simulink library "sf_pole_vault_lib"  (R2025b)
settings: Solver=VariableStepAuto  StartTime=0.0  StopTime=10.0  RelTol=1e-3
undefined symbols (not defined in the file or in its folder): theta0
libraries: simulink_extras x3
settings Model: Creator=The MathWorks, Inc.  LastModifiedBy=The MathWorks, Inc.
settings SolverCC: AlgebraicLoopSolver=TrustRegion
settings DataIOCC: ReturnWorkspaceOutputs=off
settings OptimizationCC: ReuseModelBlockBuffer=off
settings DebuggingCC: UnconnectedInputMsg=warning  UnconnectedOutputMsg=warning  UnconnectedLineMsg=warning  ArithmeticOperatorsInVariantConditions=warning
settings ModelReferenceCC: EnableRefExpFcnMdlSchedulingChecks=on
settings SFSimCC: SimUseLocalCustomCode=off  CustomCodeUndefinedFunction=UseInterfaceOnly
settings RTWCC: RTWUseLocalCustomCode=off  GPUComputeCapability=3.5

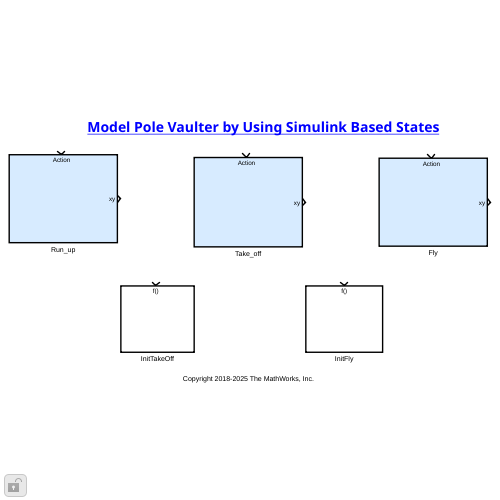
[thumbnail: Simulink's stored preview of the top-level diagram]
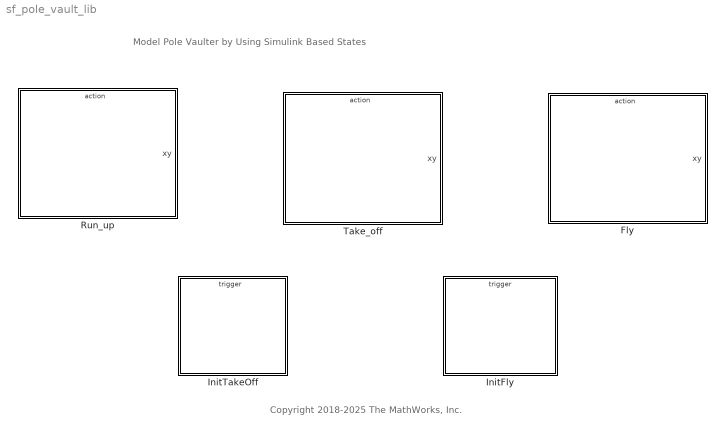
== system sf_pole_vault_lib ==
  note: Copyright 2018-2025 The MathWorks, Inc.
  note: Model Pole Vaulter by Using Simulink Based States
  Fly : Subsystem
      settings: UndoDeleteFcn=Stateflow.SLINSF.SimulinkMan.restorePreDeleteFcn  PreDeleteFcn=Stateflow.SLINSF.SimulinkMan.removePreDeleteFcn
  InitFly : Subsystem
      settings: UndoDeleteFcn=Stateflow.SLINSF.SimulinkMan.restorePreDeleteFcn  PreDeleteFcn=Stateflow.SLINSF.SimulinkMan.removePreDeleteFcn
  InitTakeOff : Subsystem
      settings: UndoDeleteFcn=Stateflow.SLINSF.SimulinkMan.restorePreDeleteFcn  PreDeleteFcn=Stateflow.SLINSF.SimulinkMan.removePreDeleteFcn
  Run_up : Subsystem
      settings: UndoDeleteFcn=Stateflow.SLINSF.SimulinkMan.restorePreDeleteFcn  PreDeleteFcn=Stateflow.SLINSF.SimulinkMan.removePreDeleteFcn
  Take_off : Subsystem
      settings: UndoDeleteFcn=Stateflow.SLINSF.SimulinkMan.restorePreDeleteFcn  PreDeleteFcn=Stateflow.SLINSF.SimulinkMan.removePreDeleteFcn

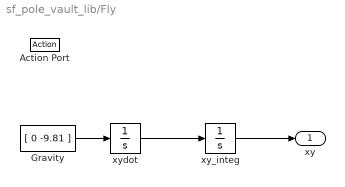
== system sf_pole_vault_lib/Fly ==
  Action Port : ActionPort
      settings: CopyFcn=Stateflow.SLINSF.SimulinkMan.removeBlockPreDeleteFcn
  Gravity : Constant  Value=[ 0 -9.81 ]
  xy_integ : Integrator
  xydot : Integrator
  xy : Outport  VectorParamsAs1DForOutWhenUnconnected=off
  wires:
  xy_integ/1 -> xy/1
  xydot/1 -> xy_integ/1
  Gravity/1 -> xydot/1

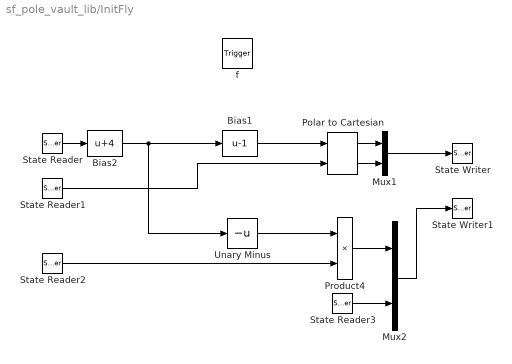
== system sf_pole_vault_lib/InitFly ==
  f : TriggerPort  TriggerType=function-call  VariantControl=Variant
      settings: CopyFcn=Stateflow.SLINSF.SimulinkMan.removeBlockPreDeleteFcn
  Bias1 : Bias  Bias=-1  SaturateOnIntegerOverflow=off
  Bias2 : Bias  Bias=4  SaturateOnIntegerOverflow=off
  Mux1 : Mux  Inputs=2
  Mux2 : Mux  Inputs=2
  Polar to Cartesian : simulink_extras/Transformations/Polar to Cartesian
  Product4 : Product
  State Reader : StateReader  StateOwnerBlock=../../Take_off/r  StateName=r
  State Reader1 : StateReader  StateOwnerBlock=../../Take_off/theta  StateName=theta
  State Reader2 : StateReader  StateOwnerBlock=../../Take_off/theta_dot  StateName=theta_dot
  State Reader3 : StateReader  StateOwnerBlock=../../Take_off/r_dot  StateName=rdot
  State Writer : StateWriter  StateOwnerBlock=../../Fly/xy_integ
  State Writer1 : StateWriter  StateOwnerBlock=../../Fly/xydot
  Unary Minus : UnaryMinus
  wires:
  Unary Minus/1 -> Product4/1
  Bias2/1 -> Bias1/1, Unary Minus/1
  State Reader3/1 -> Mux2/2
  State Reader2/1 -> Product4/2
  Polar to Cartesian/2 -> Mux1/2
  Product4/1 -> Mux2/1
  Bias1/1 -> Polar to Cartesian/1
  State Reader/1 -> Bias2/1
  State Reader1/1 -> Polar to Cartesian/2
  Polar to Cartesian/1 -> Mux1/1
  Mux2/1 -> State Writer1/1
  Mux1/1 -> State Writer/1

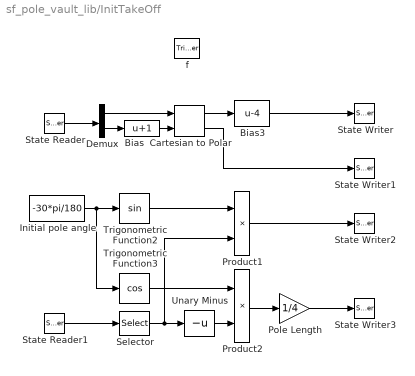
== system sf_pole_vault_lib/InitTakeOff ==
  f : TriggerPort  TriggerType=function-call  VariantControl=Variant
      settings: CopyFcn=Stateflow.SLINSF.SimulinkMan.removeBlockPreDeleteFcn
  Bias : Bias  Bias=1  SaturateOnIntegerOverflow=off
  Bias3 : Bias  Bias=-4  SaturateOnIntegerOverflow=off
  Cartesian to Polar : simulink_extras/Transformations/Cartesian to Polar
  Demux : Demux  Outputs=2
  Initial pole angle : Constant  Value=-30*pi/180
  Pole Length : Gain  Gain=1/4
  Product1 : Product
  Product2 : Product
  Selector : Selector  InputPortWidth=2  IndexOptions=Index vector (dialog)  Indices=1  OutputSizes=1
  State Reader : StateReader  StateOwnerBlock=../../Run_up/Position  StateName=p
  State Reader1 : StateReader  StateOwnerBlock=../../Run_up/Velocity  StateName=v
  State Writer : StateWriter  StateOwnerBlock=../../Take_off/r  StateName=r
  State Writer1 : StateWriter  StateOwnerBlock=../../Take_off/theta  StateName=theta
  State Writer2 : StateWriter  StateOwnerBlock=../../Take_off/r_dot  StateName=rdot
  State Writer3 : StateWriter  StateOwnerBlock=../../Take_off/theta_dot  StateName=theta_dot
  Trigonometric Function2 : Trigonometry
  Trigonometric Function3 : Trigonometry  Operator=cos
  Unary Minus : UnaryMinus
  wires:
  Demux/1 -> Cartesian to Polar/1
  Initial pole angle/1 -> Trigonometric Function2/1, Trigonometric Function3/1
  Pole Length/1 -> State Writer3/1
  Product2/1 -> Pole Length/1
  State Reader1/1 -> Selector/1
  Cartesian to Polar/2 -> State Writer1/1
  State Reader/1 -> Demux/1
  Bias/1 -> Cartesian to Polar/2
  Cartesian to Polar/1 -> Bias3/1
  Demux/2 -> Bias/1
  Product1/1 -> State Writer2/1
  Trigonometric Function2/1 -> Product1/1
  Selector/1 -> Unary Minus/1, Product1/2
  Bias3/1 -> State Writer/1
  Trigonometric Function3/1 -> Product2/1
  Unary Minus/1 -> Product2/2

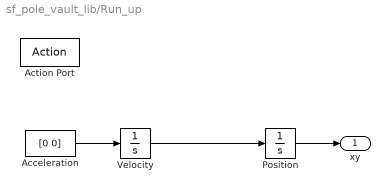
== system sf_pole_vault_lib/Run_up ==
  Action Port : ActionPort
      settings: CopyFcn=Stateflow.SLINSF.SimulinkMan.removeBlockPreDeleteFcn
  Acceleration : Constant  Value=[0 0]
  Position : Integrator  InitialCondition=[-10 0.1]  ContinuousStateAttributes='p'
      settings: AttributesFormatString=x0 = %<InitialCondition>
  Velocity : Integrator  InitialCondition=[15 0]  ContinuousStateAttributes='v'
      settings: AttributesFormatString=v0 = %<InitialCondition>
  xy : Outport  VectorParamsAs1DForOutWhenUnconnected=off
  wires:
  Velocity/1 -> Position/1
  Acceleration/1 -> Velocity/1
  Position/1 -> xy/1

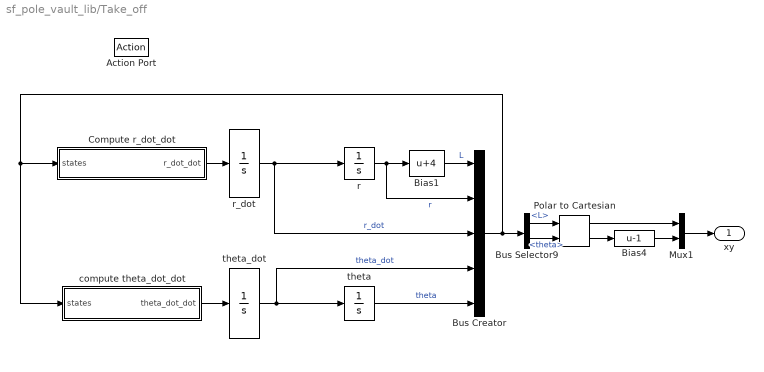
== system sf_pole_vault_lib/Take_off ==
  Action Port : ActionPort
      settings: CopyFcn=Stateflow.SLINSF.SimulinkMan.removeBlockPreDeleteFcn
  Bias1 : Bias  Bias=4  SaturateOnIntegerOverflow=off
  Bias4 : Bias  Bias=-1  SaturateOnIntegerOverflow=off
  Bus Creator : BusCreator  Inputs=5
  Bus Selector9 : BusSelector  OutputSignals=L,theta
  Compute r_dot_dot : Subsystem
  Mux1 : Mux  Inputs=2
  Polar to Cartesian : simulink_extras/Transformations/Polar to Cartesian
  compute theta_dot_dot : Subsystem
  r : Integrator  ContinuousStateAttributes='r'
  r_dot : Integrator  InitialCondition=-10*sin(30*pi/180)  ContinuousStateAttributes='rdot'
  theta : Integrator  InitialCondition=theta0  ContinuousStateAttributes='theta'
  theta_dot : Integrator  InitialCondition=10*cos(30*pi/180)/4  ContinuousStateAttributes='theta_dot'
  xy : Outport  VectorParamsAs1DForOutWhenUnconnected=off
  wires:
  compute theta_dot_dot/1(theta_dot_dot) -> theta_dot/1
  Compute r_dot_dot/1(r_dot_dot) -> r_dot/1
  Bias4/1 -> Mux1/2
  Polar to Cartesian/1 -> Mux1/1
  Bus Selector9/2 -> Polar to Cartesian/2  "<theta>"
  Bus Selector9/1 -> Polar to Cartesian/1  "<L>"
  theta/1 -> Bus Creator/5  "theta"
  Polar to Cartesian/2 -> Bias4/1
  Mux1/1 -> xy/1
  Bus Creator/1 -> Compute r_dot_dot/1(states), compute theta_dot_dot/1(states), Bus Selector9/1
  Bias1/1 -> Bus Creator/1  "L"
  theta_dot/1 -> theta/1, Bus Creator/4  "theta_dot"
  r/1 -> Bias1/1, Bus Creator/2  "r"
  r_dot/1 -> r/1, Bus Creator/3  "r_dot"

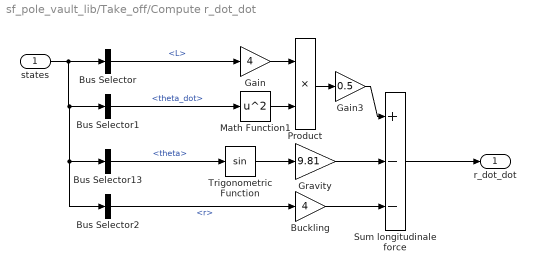
== system sf_pole_vault_lib/Take_off/Compute r_dot_dot ==
  states : Inport
  Buckling : Gain  Gain=4
  Bus Selector : BusSelector  OutputSignals=L
  Bus Selector1 : BusSelector  OutputSignals=theta_dot
  Bus Selector13 : BusSelector  OutputSignals=theta
  Bus Selector2 : BusSelector  OutputSignals=r
  Gain : Gain  Gain=4
  Gain3 : Gain  Gain=0.5
  Gravity : Gain  Gain=9.81
  Math Function1 : Math  Operator=square  SignedPower=on
  Product : Product
  Sum longitudinale force : Sum  Inputs=+--
  Trigonometric Function : Trigonometry
  r_dot_dot : Outport  VectorParamsAs1DForOutWhenUnconnected=off
  wires:
  Bus Selector13/1 -> Trigonometric Function/1  "<theta>"
  states/1 -> Bus Selector/1, Bus Selector1/1, Bus Selector13/1, Bus Selector2/1
  Sum longitudinale force/1 -> r_dot_dot/1
  Math Function1/1 -> Product/2
  Product/1 -> Gain3/1
  Trigonometric Function/1 -> Gravity/1
  Buckling/1 -> Sum longitudinale force/3
  Gravity/1 -> Sum longitudinale force/2
  Gain/1 -> Product/1
  Gain3/1 -> Sum longitudinale force/1
  Bus Selector1/1 -> Math Function1/1  "<theta_dot>"
  Bus Selector/1 -> Gain/1  "<L>"
  Bus Selector2/1 -> Buckling/1  "<r>"

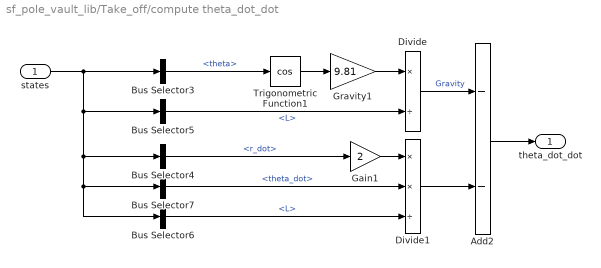
== system sf_pole_vault_lib/Take_off/compute theta_dot_dot ==
  states : Inport
  Add2 : Sum  Inputs=--
  Bus Selector3 : BusSelector  OutputSignals=theta
  Bus Selector4 : BusSelector  OutputSignals=r_dot
  Bus Selector5 : BusSelector  OutputSignals=L
  Bus Selector6 : BusSelector  OutputSignals=L
  Bus Selector7 : BusSelector  OutputSignals=theta_dot
  Divide : Product  Inputs=*/
  Divide1 : Product  Inputs=**/
  Gain1 : Gain  Gain=2
  Gravity1 : Gain  Gain=9.81
  Trigonometric Function1 : Trigonometry  Operator=cos
  theta_dot_dot : Outport  VectorParamsAs1DForOutWhenUnconnected=off
  wires:
  Gravity1/1 -> Divide/1
  states/1 -> Bus Selector3/1, Bus Selector4/1, Bus Selector7/1, Bus Selector6/1, Bus Selector5/1
  Add2/1 -> theta_dot_dot/1
  Gain1/1 -> Divide1/1
  Divide/1 -> Add2/1  "Gravity"
  Divide1/1 -> Add2/2
  Trigonometric Function1/1 -> Gravity1/1
  Bus Selector7/1 -> Divide1/2  "<theta_dot>"
  Bus Selector5/1 -> Divide/2  "<L>"
  Bus Selector6/1 -> Divide1/3  "<L>"
  Bus Selector4/1 -> Gain1/1  "<r_dot>"
  Bus Selector3/1 -> Trigonometric Function1/1  "<theta>"
